simulink model "geometric_control_pertub"  (R2025b)
settings: Solver=ode45  StartTime=0.0  StopTime=t(end)  MaxStep=Ts  RelTol=1e-5
values from neighbouring files (symbols this model uses):
  A_tau = 0.002    [disturbances.m]    (also in scenarios_dist.m = K_dist * A_tau)
  A_wind = 0.1    [disturbances.m]    (also in scenarios_dist.m = K_dist * A_wind)
  Awind_0 = 0.5    [disturbances.m]    (also in scenarios_dist.m = K_dist * Awind_0)
  c_plant = 40/epsilon    (= 40)    [data.m]    (also in variation_params.m = scenarios(scen_idx, 2))
  Cd_eta = [0.08; 0.08; 0.05; 0.1; 0.1]    [disturbances.m]
  Cd_gamma = [0.01; 0.01; 0.01]    [disturbances.m]
  Cv_eta = [0.3; 0.3; 0.15; 0.4; 0.4]    [disturbances.m]
  Cv_gamma = [0.05; 0.05; 0.02]    [disturbances.m]
  dot_q_0 = -(dot_A_0 - (q_0' * dot_A_0) * q_0) / norm_A0    [trajectory_smooth.m]
  J = diag([Ixx, Iyy, Izz])    [data.m]
  k_plant = 1e5/epsilon^2    (= 100000)    [data.m]    (also in variation_params.m = scenarios(scen_idx, 1))
  kdq = 15    [control_params.m]
  kdw = 0.05    [disturbances.m]
  kO = 5    [control_params.m]
  kq = 50    [control_params.m]
  kr = 15    [control_params.m]
  kv = 15    [control_params.m]
  kx = 35    [control_params.m]
  L = 1    [data.m]
  l_0 = L + (m_L_plant * norm_A0) / (k_plant*m_sum_plant)    [trajectory_smooth.m]
  m_L = 0.5    [data.m]
  m_L_plant = m_L    (= 0.5)    [data.m]    (also in variation_params.m = scenarios(scen_idx, 3))
  m_q = 2    [data.m]
  Omega_0 = [0; 0; 0]    [trajectory_smooth.m]
  omega_0 = cross(q_0, dot_q_0)    [trajectory_smooth.m]
  omega_n_1 = 50    [control_params.m]
  omega_n_2 = 100    [control_params.m]
  omg_w = 0.8    [disturbances.m]
  q_0 = -A_0 / norm_A0    [trajectory_smooth.m]
  R_0 = [b1_0, b2_0, b3_0]    [trajectory_smooth.m]
  tau_phi_0 = 0.01    [disturbances.m]    (also in scenarios_dist.m = K_dist * tau_phi_0)
  tau_psi_0 = 0.005    [disturbances.m]    (also in scenarios_dist.m = K_dist * tau_psi_0)
  tau_theta_0 = 0.01    [disturbances.m]    (also in scenarios_dist.m = K_dist * tau_theta_0)
  vl_0 = dot_csi_d(:, 1)    [trajectory_smooth.m]
  xl_0 = csi_d(:, 1)    [trajectory_smooth.m]
  zeta_1 = 1    [control_params.m]
  zeta_2 = zeta_1    (= 1)    [control_params.m]
settings Model: Creator=emanu  LastModifiedBy=emanu

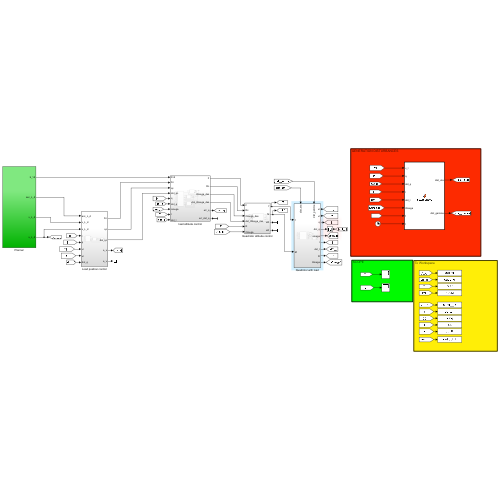
[thumbnail: Simulink's stored preview of the top-level diagram]
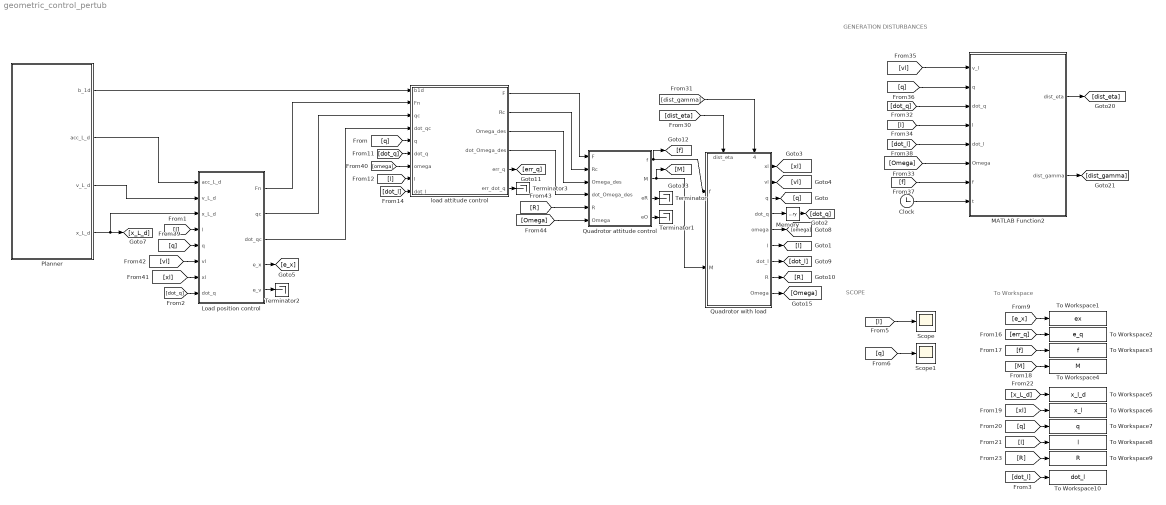
== system geometric_control_pertub ==
  note: GENERATION DISTURBANCES
  note: To Workspace
  note: SCOPE
  Clock : Clock
  Load position control : Subsystem
  MATLAB Function2 : MATLAB Function  TreatAsAtomicUnit=on
  Memory : Memory  InitialCondition=dot_q_0
  Planner : Subsystem
  Quadrotor attitude control : Subsystem
  Quadrotor with load : Subsystem
      settings: PortSchema="{\"entries\":[{\"content\":{\"sides\":[{\"content\":{\"connectorIds\":[\"In1\",\"In2\"]},\"type\":\"ConnectorPlacement.EquallySpacedRectSide\",\"uuid\":\"bde89180-b818-445b-bc24-a963d30a6ca2\"},{\"content\":{\"connectorIds\":[\"Out1\",\"Out2\",\"Out3\",\"Out4\",\"Out5\",\"Out6\",\"Out7\",\"Out8\",\"Out9\"],\"side\":\"RIGHT\"},\"type\":\"ConnectorPlacement.EquallySpacedRectSide\",\"uuid\":\"01dfe049-2eac-475a-b8e9-907eef5903e1\"},{\"content\":{\"connectorIds\":[\"In3\",\"In4\"],\"side\":\"TOP\"},\"type\":\"ConnectorPlacement.EquallySpacedRectSide\",\"uuid\":\"9cbb9b96-1170-48a0-bc43-4ca5d32b1acc\"}]},\"type\":\"ConnectorPlacement.EquallySpacedConnector\",\"uuid\":\"6cb2dbf7-60ad-42b8-8943-1cecbded3d22\"}],\"packageUris\":[\"http://schema.mathworks.com/mf0/Connector/R2020b\"],\"version\":\"1.0\"}"
  Scope : Scope
      settings: ActiveDisplayYMinimum=-1  ActiveDisplayYMaximum=1
  Scope1 : Scope
  Terminator{,1..3} (4 alike) : Terminator
  To Workspace1 : ToWorkspace  VariableName=ex  SaveFormat=Timeseries  SampleTime=-1
  To Workspace10 : ToWorkspace  VariableName=dot_l  SaveFormat=Timeseries  SampleTime=-1
  To Workspace2 : ToWorkspace  VariableName=e_q  SaveFormat=Timeseries  SampleTime=-1
  To Workspace3 : ToWorkspace  VariableName=f  SaveFormat=Timeseries  SampleTime=-1
  To Workspace4 : ToWorkspace  VariableName=M  SaveFormat=Timeseries  SampleTime=-1
  To Workspace5 : ToWorkspace  VariableName=x_l_d  SaveFormat=Timeseries  SampleTime=-1
  To Workspace6 : ToWorkspace  VariableName=x_l  SaveFormat=Timeseries  SampleTime=-1
  To Workspace7 : ToWorkspace  VariableName=q  SaveFormat=Timeseries  SampleTime=-1
  To Workspace8 : ToWorkspace  VariableName=l  SaveFormat=Timeseries  SampleTime=-1
  To Workspace9 : ToWorkspace  VariableName=R  SaveFormat=Timeseries  SampleTime=-1
  load attitude control : Subsystem
  wires:
  Quadrotor attitude control/1(f) -> [f], Quadrotor with load/1(f)
  Quadrotor attitude control/2(M) -> Quadrotor with load/2(M), [M]
  Quadrotor attitude control/3(eR) -> Terminator/1
  Quadrotor attitude control/4(eO) -> Terminator1/1
  load attitude control/1(F) -> Quadrotor attitude control/1(F)
  load attitude control/2(Rc) -> Quadrotor attitude control/2(Rc)
  load attitude control/3(Omega_des) -> Quadrotor attitude control/3(Omega_des)
  load attitude control/4(dot_Omega_des) -> Quadrotor attitude control/4(dot_Omega_des)
  Load position control/1(Fn) -> load attitude control/2(Fn)
  Load position control/2(qc) -> load attitude control/3(qc)
  Load position control/3(dot_qc) -> load attitude control/4(dot_qc)
  [l] -> Load position control/4(l)
  [dot_q] -> Load position control/8(dot_q)
  load attitude control/5(err_q) -> [err_q]
  load attitude control/6(err_dot_q) -> Terminator3/1
  Planner/1(b_1d) -> load attitude control/1(b1d)
  Planner/2(acc_L_d) -> Load position control/1(acc_L_d)
  Planner/3(v_L_d) -> Load position control/2(v_L_d)
  Planner/4(x_L_d) -> [x_L_d], Load position control/3(x_L_d)
  Quadrotor with load/6(l) -> [l]
  Quadrotor with load/5(omega) -> [omega]
  Quadrotor with load/3(q) -> [q]
  Quadrotor with load/1(xl) -> [xl]
  Quadrotor with load/2(vl) -> [vl]
  Load position control/4(e_x) -> [e_x]
  Load position control/5(e_v) -> Terminator2/1
  Memory/1 -> [dot_q]
  Quadrotor with load/4(dot_q) -> Memory/1
  [dot_q] -> load attitude control/6(dot_q)
  [l] -> load attitude control/8(l)
  Quadrotor with load/7(dot_l) -> [dot_l]
  [dot_l] -> load attitude control/9(dot_l)
  Quadrotor with load/8(R) -> [R]
  [e_x] -> To Workspace1/1
  [err_q] -> To Workspace2/1
  [f] -> To Workspace3/1
  [M] -> To Workspace4/1
  [x_L_d] -> To Workspace5/1
  [xl] -> To Workspace6/1
  [q] -> To Workspace7/1
  [l] -> To Workspace8/1
  [R] -> To Workspace9/1
  [l] -> Scope/1
  [q] -> Scope1/1
  Quadrotor with load/9(Omega) -> [Omega]
  MATLAB Function2/1(dist_eta) -> [dist_eta]
  MATLAB Function2/2(dist_gamma) -> [dist_gamma]
  [dist_eta] -> Quadrotor with load/3(dist_eta)
  [dist_gamma] -> Quadrotor with load/4(dist_gamma)
  [l] -> MATLAB Function2/4(l)
  [dot_q] -> MATLAB Function2/3(dot_q)
  [vl] -> MATLAB Function2/1(v_l)
  Clock/1 -> MATLAB Function2/8(t)
  [Omega] -> MATLAB Function2/6(Omega)
  [q] -> MATLAB Function2/2(q)
  [f] -> MATLAB Function2/7(f)
  [dot_l] -> MATLAB Function2/5(dot_l)
  [q] -> Load position control/5(q)
  [omega] -> load attitude control/7(omega)
  [xl] -> Load position control/7(xl)
  [vl] -> Load position control/6(vl)
  [R] -> Quadrotor attitude control/5(R)
  [Omega] -> Quadrotor attitude control/6(Omega)
  [q] -> load attitude control/5(q)
  [dot_l] -> To Workspace10/1

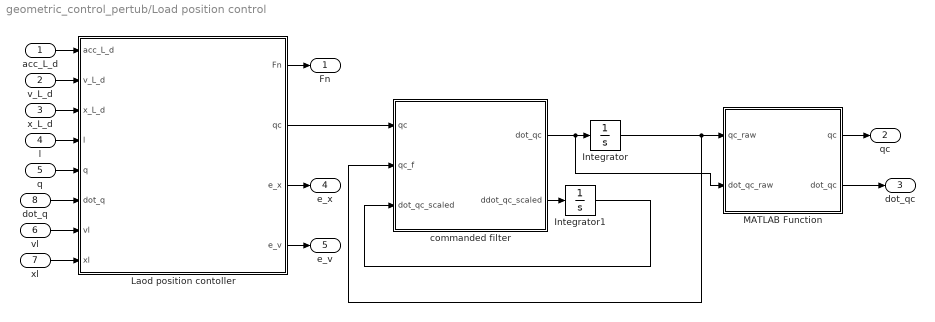
== system geometric_control_pertub/Load position control ==
  acc_L_d : Inport
  v_L_d : Inport  Port=2
  x_L_d : Inport  Port=3
  l : Inport  Port=4
  q : Inport  Port=5
  vl : Inport  Port=6
  xl : Inport  Port=7
  dot_q : Inport  Port=8
  Integrator : Integrator  InitialCondition=q_0
  Integrator1 : Integrator  InitialCondition=dot_q_0
  Laod position contoller : MATLAB Function  TreatAsAtomicUnit=on
  MATLAB Function : MATLAB Function  TreatAsAtomicUnit=on
  commanded filter : MATLAB Function  TreatAsAtomicUnit=on
  Fn : Outport
  qc : Outport  Port=2
  dot_qc : Outport  Port=3
  e_x : Outport  Port=4  VectorParamsAs1DForOutWhenUnconnected=off
  e_v : Outport  Port=5  VectorParamsAs1DForOutWhenUnconnected=off
  wires:
  acc_L_d/1 -> Laod position contoller/1(acc_L_d)
  v_L_d/1 -> Laod position contoller/2(v_L_d)
  x_L_d/1 -> Laod position contoller/3(x_L_d)
  l/1 -> Laod position contoller/4(l)
  q/1 -> Laod position contoller/5(q)
  vl/1 -> Laod position contoller/7(vl)
  xl/1 -> Laod position contoller/8(xl)
  Laod position contoller/1(Fn) -> Fn/1
  Laod position contoller/2(qc) -> commanded filter/1(qc)
  dot_q/1 -> Laod position contoller/6(dot_q)
  Laod position contoller/3(e_x) -> e_x/1
  Laod position contoller/4(e_v) -> e_v/1
  commanded filter/1(dot_qc) -> MATLAB Function/2(dot_qc_raw), Integrator/1
  Integrator/1 -> MATLAB Function/1(qc_raw), commanded filter/2(qc_f)
  commanded filter/2(ddot_qc_scaled) -> Integrator1/1
  Integrator1/1 -> commanded filter/3(dot_qc_scaled)
  MATLAB Function/1(qc) -> qc/1
  MATLAB Function/2(dot_qc) -> dot_qc/1

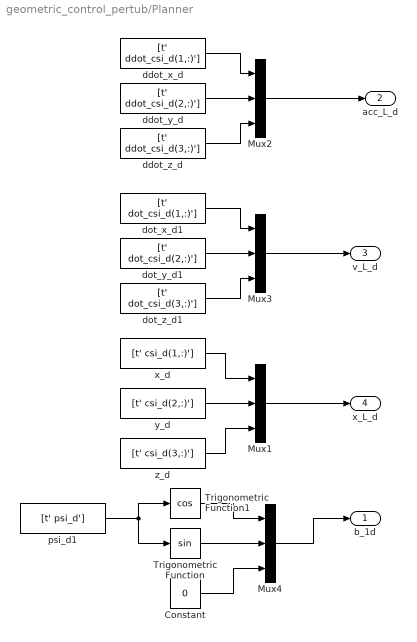
== system geometric_control_pertub/Planner ==
  Constant : Constant  Value=0
  Mux{1..4} (4 alike) : Mux  Inputs=3
  Trigonometric Function : Trigonometry
  Trigonometric Function1 : Trigonometry  Operator=cos
  ddot_x_d : FromWorkspace  VariableName=[t' ddot_csi_d(1,:)']  OutputAfterFinalValue=Holding final value
  ddot_y_d : FromWorkspace  VariableName=[t' ddot_csi_d(2,:)']  OutputAfterFinalValue=Holding final value
  ddot_z_d : FromWorkspace  VariableName=[t' ddot_csi_d(3,:)']  OutputAfterFinalValue=Holding final value
  dot_x_d1 : FromWorkspace  VariableName=[t' dot_csi_d(1,:)']  OutputAfterFinalValue=Holding final value
  dot_y_d1 : FromWorkspace  VariableName=[t' dot_csi_d(2,:)']  OutputAfterFinalValue=Holding final value
  dot_z_d1 : FromWorkspace  VariableName=[t' dot_csi_d(3,:)']  OutputAfterFinalValue=Holding final value
  psi_d1 : FromWorkspace  VariableName=[t' psi_d']  OutputAfterFinalValue=Holding final value
  x_d : FromWorkspace  VariableName=[t' csi_d(1,:)']  OutputAfterFinalValue=Holding final value
  y_d : FromWorkspace  VariableName=[t' csi_d(2,:)']  OutputAfterFinalValue=Holding final value
  z_d : FromWorkspace  VariableName=[t' csi_d(3,:)']  OutputAfterFinalValue=Holding final value
  b_1d : Outport
  acc_L_d : Outport  Port=2
  v_L_d : Outport  Port=3
  x_L_d : Outport  Port=4
  wires:
  y_d/1 -> Mux1/2
  z_d/1 -> Mux1/3
  x_d/1 -> Mux1/1
  ddot_y_d/1 -> Mux2/2
  ddot_z_d/1 -> Mux2/3
  ddot_x_d/1 -> Mux2/1
  Mux2/1 -> acc_L_d/1
  Mux1/1 -> x_L_d/1
  dot_y_d1/1 -> Mux3/2
  dot_z_d1/1 -> Mux3/3
  dot_x_d1/1 -> Mux3/1
  Mux3/1 -> v_L_d/1
  Mux4/1 -> b_1d/1
  Trigonometric Function/1 -> Mux4/2
  psi_d1/1 -> Trigonometric Function/1, Trigonometric Function1/1
  Trigonometric Function1/1 -> Mux4/1
  Constant/1 -> Mux4/3

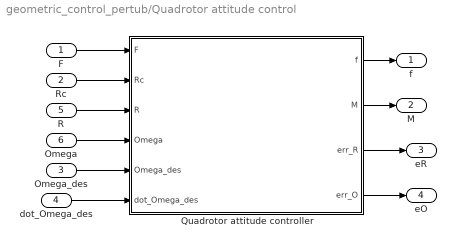
== system geometric_control_pertub/Quadrotor attitude control ==
  F : Inport
  Rc : Inport  Port=2
  Omega_des : Inport  Port=3
  dot_Omega_des : Inport  Port=4
  R : Inport  Port=5
  Omega : Inport  Port=6
  Quadrotor attitude controller : MATLAB Function  TreatAsAtomicUnit=on
  f : Outport
  M : Outport  Port=2
  eR : Outport  Port=3
  eO : Outport  Port=4
  wires:
  F/1 -> Quadrotor attitude controller/1(F)
  Quadrotor attitude controller/1(f) -> f/1
  Quadrotor attitude controller/2(M) -> M/1
  Quadrotor attitude controller/3(err_R) -> eR/1
  Quadrotor attitude controller/4(err_O) -> eO/1
  R/1 -> Quadrotor attitude controller/3(R)
  Omega/1 -> Quadrotor attitude controller/4(Omega)
  Omega_des/1 -> Quadrotor attitude controller/5(Omega_des)
  dot_Omega_des/1 -> Quadrotor attitude controller/6(dot_Omega_des)
  Rc/1 -> Quadrotor attitude controller/2(Rc)

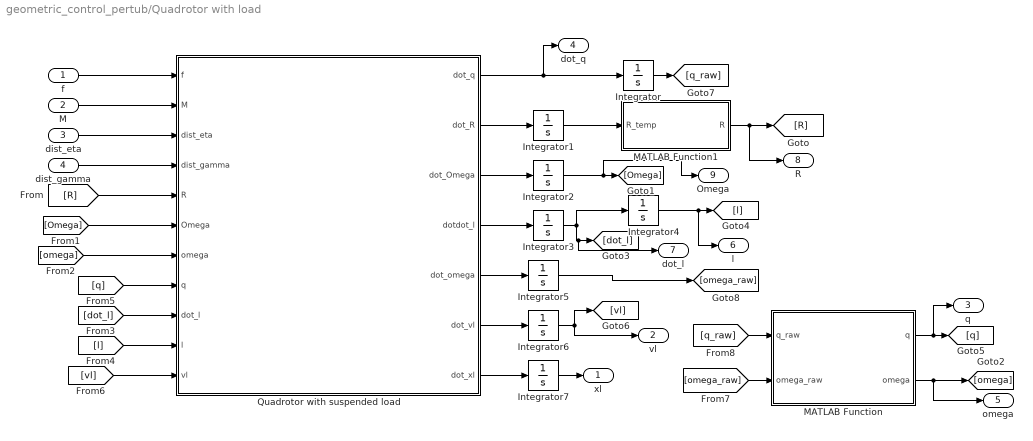
== system geometric_control_pertub/Quadrotor with load ==
  f : Inport
  M : Inport  Port=2
  dist_eta : Inport  Port=3
  dist_gamma : Inport  Port=4
  Integrator : Integrator  InitialCondition=q_0
  Integrator1 : Integrator  InitialCondition=R_0
  Integrator2 : Integrator  InitialCondition=Omega_0
  Integrator3 : Integrator
  Integrator4 : Integrator  InitialCondition=l_0
  Integrator5 : Integrator  InitialCondition=omega_0
  Integrator6 : Integrator  InitialCondition=vl_0
  Integrator7 : Integrator  InitialCondition=xl_0
  MATLAB Function : MATLAB Function  TreatAsAtomicUnit=on
  MATLAB Function1 : MATLAB Function  TreatAsAtomicUnit=on
  "Quadrotor with suspended load " : MATLAB Function  TreatAsAtomicUnit=on
  xl : Outport
  vl : Outport  Port=2
  q : Outport  Port=3
  dot_q : Outport  Port=4
  omega : Outport  Port=5
  l : Outport  Port=6
  dot_l : Outport  Port=7
  R : Outport  Port=8
  Omega : Outport  Port=9
  wires:
  f/1 -> "Quadrotor with suspended load "/1(f)
  M/1 -> "Quadrotor with suspended load "/2(M)
  "Quadrotor with suspended load "/1(dot_q) -> dot_q/1, Integrator/1
  "Quadrotor with suspended load "/2(dot_R) -> Integrator1/1
  Integrator1/1 -> MATLAB Function1/1(R_temp)
  MATLAB Function1/1(R) -> R/1, [R]
  [R] -> "Quadrotor with suspended load "/5(R)
  "Quadrotor with suspended load "/3(dot_Omega) -> Integrator2/1
  Integrator2/1 -> Omega/1, [Omega]
  [Omega] -> "Quadrotor with suspended load "/6(Omega)
  "Quadrotor with suspended load "/4(dotdot_l) -> Integrator3/1
  Integrator3/1 -> Integrator4/1, dot_l/1, [dot_l]
  "Quadrotor with suspended load "/5(dot_omega) -> Integrator5/1
  [omega] -> "Quadrotor with suspended load "/7(omega)
  [dot_l] -> "Quadrotor with suspended load "/9(dot_l)
  Integrator4/1 -> l/1, [l]
  [l] -> "Quadrotor with suspended load "/10(l)
  [q] -> "Quadrotor with suspended load "/8(q)
  "Quadrotor with suspended load "/6(dot_vl) -> Integrator6/1
  Integrator6/1 -> [vl], vl/1
  [vl] -> "Quadrotor with suspended load "/11(vl)
  "Quadrotor with suspended load "/7(dot_xl) -> Integrator7/1
  Integrator7/1 -> xl/1
  Integrator/1 -> [q_raw]
  Integrator5/1 -> [omega_raw]
  [omega_raw] -> MATLAB Function/2(omega_raw)
  [q_raw] -> MATLAB Function/1(q_raw)
  MATLAB Function/1(q) -> q/1, [q]
  MATLAB Function/2(omega) -> omega/1, [omega]
  dist_eta/1 -> "Quadrotor with suspended load "/3(dist_eta)
  dist_gamma/1 -> "Quadrotor with suspended load "/4(dist_gamma)

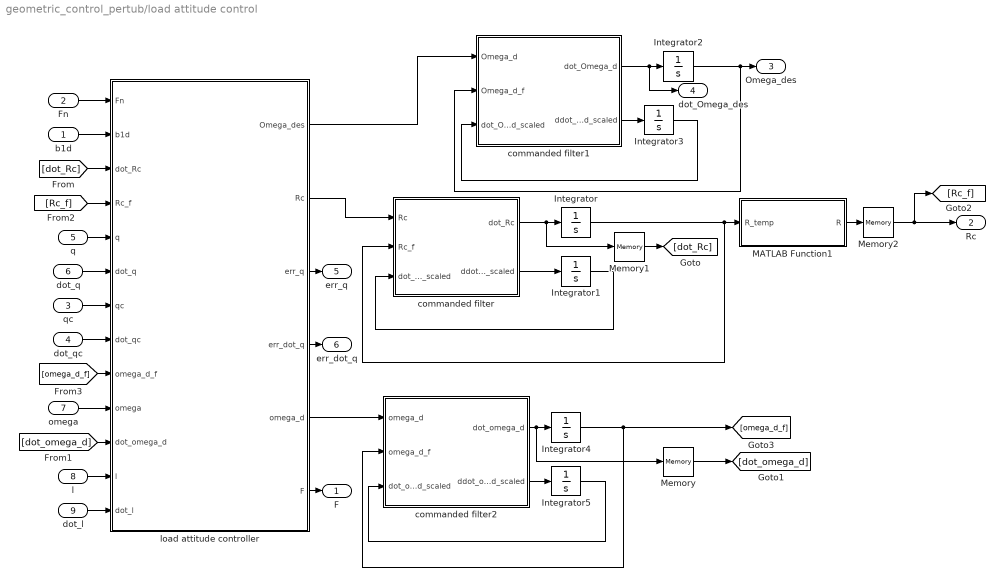
== system geometric_control_pertub/load attitude control ==
  b1d : Inport
  Fn : Inport  Port=2
  qc : Inport  Port=3
  dot_qc : Inport  Port=4
  q : Inport  Port=5
  dot_q : Inport  Port=6
  omega : Inport  Port=7
  l : Inport  Port=8
  dot_l : Inport  Port=9
  Integrator : Integrator  InitialCondition=R_0
  Integrator1 : Integrator  InitialCondition=zeros(3,3)
  Integrator2 : Integrator  InitialCondition=Omega_0
  Integrator3 : Integrator  InitialCondition=zeros(3,1)
  Integrator4 : Integrator  InitialCondition=omega_0
  Integrator5 : Integrator  InitialCondition=zeros(3,1)
  MATLAB Function1 : MATLAB Function  TreatAsAtomicUnit=on
  Memory : Memory  InitialCondition=zeros(3,1)
  Memory1 : Memory  InitialCondition=zeros(3,3)
  Memory2 : Memory  InitialCondition=R_0
  commanded filter : MATLAB Function  TreatAsAtomicUnit=on
  commanded filter1 : MATLAB Function  TreatAsAtomicUnit=on
  commanded filter2 : MATLAB Function  TreatAsAtomicUnit=on
  load attitude controller : MATLAB Function  TreatAsAtomicUnit=on
  F : Outport
  Rc : Outport  Port=2
  Omega_des : Outport  Port=3
  dot_Omega_des : Outport  Port=4
  err_q : Outport  Port=5  VectorParamsAs1DForOutWhenUnconnected=off
  err_dot_q : Outport  Port=6
  wires:
  load attitude controller/2(Rc) -> commanded filter/1(Rc)
  [dot_Rc] -> load attitude controller/3(dot_Rc)
  Integrator5/1 -> commanded filter2/3(dot_omega_d_scaled)
  [dot_omega_d] -> load attitude controller/11(dot_omega_d)
  qc/1 -> load attitude controller/7(qc)
  dot_qc/1 -> load attitude controller/8(dot_qc)
  q/1 -> load attitude controller/5(q)
  dot_q/1 -> load attitude controller/6(dot_q)
  omega/1 -> load attitude controller/10(omega)
  l/1 -> load attitude controller/12(l)
  dot_l/1 -> load attitude controller/13(dot_l)
  load attitude controller/6(F) -> F/1
  b1d/1 -> load attitude controller/2(b1d)
  Fn/1 -> load attitude controller/1(Fn)
  load attitude controller/3(err_q) -> err_q/1
  load attitude controller/4(err_dot_q) -> err_dot_q/1
  commanded filter/1(dot_Rc) -> Memory1/1, Integrator/1
  Integrator1/1 -> commanded filter/3(dot_Rc_scaled)
  Integrator/1 -> commanded filter/2(Rc_f), MATLAB Function1/1(R_temp)
  commanded filter/2(ddot_Rc_scaled) -> Integrator1/1
  commanded filter2/2(ddot_omega_d_scaled) -> Integrator5/1
  commanded filter2/1(dot_omega_d) -> Memory/1, Integrator4/1
  load attitude controller/5(omega_d) -> commanded filter2/1(omega_d)
  commanded filter1/1(dot_Omega_d) -> dot_Omega_des/1, Integrator2/1
  commanded filter1/2(ddot_Omega_d_scaled) -> Integrator3/1
  Integrator2/1 -> Omega_des/1, commanded filter1/2(Omega_d_f)
  Integrator3/1 -> commanded filter1/3(dot_Omega_d_scaled)
  load attitude controller/1(Omega_des) -> commanded filter1/1(Omega_d)
  [Rc_f] -> load attitude controller/4(Rc_f)
  Integrator4/1 -> [omega_d_f], commanded filter2/2(omega_d_f)
  [omega_d_f] -> load attitude controller/9(omega_d_f)
  MATLAB Function1/1(R) -> Memory2/1
  Memory2/1 -> Rc/1, [Rc_f]
  Memory1/1 -> [dot_Rc]
  Memory/1 -> [dot_omega_d]

== matlab function geometric_control_pertub/Load position control/Laod position contoller ==
  data: acc_L_d input size=3; Fn output size=3; v_L_d input size=3; x_L_d input size=3; l input size=1; q input size=3; dot_q input size=3; vl input size=3; xl input size=3; qc output size=3; m_q parameter; m_L parameter; e_x output size=3; e_v output size=3; kx parameter; kv parameter
function [Fn,qc,e_x,e_v] = fcn(acc_L_d,v_L_d,x_L_d,l,q,dot_q,vl,xl,m_q, m_L,kx, kv)

g=9.81;
m_sum=m_q+m_L;
e_x=xl-x_L_d;
e_v=vl-v_L_d;

k_x =kx;
k_v = kv;

A=-k_x*e_x-k_v*e_v+m_sum*(acc_L_d+g*[0;0;1])+m_q*l*(dot_q'*dot_q)*q;
if norm(A)>1e-6
     qc=-A/norm(A);
else
    qc = [0; 0; -1];
end
Fn = (A' * q) * q;
end

== matlab function geometric_control_pertub/Quadrotor with load/MATLAB Function1 ==
  data: R_temp input; R output
function R = fcn(R_temp)
    [U,S,V] = svd(R_temp);
    sigma = det(U*V');
    S_ = diag([1 1 sigma]);

    R = U*S_*V';
end

== matlab function geometric_control_pertub/Quadrotor with load/MATLAB Function ==
  data: q_raw input; q output; omega_raw input; omega output
function [q, omega] = fcn(q_raw, omega_raw)
   
    q_raw = q_raw(:);
    omega_raw = omega_raw(:);

    
    q = q_raw / norm(q_raw);

  
    omega = omega_raw - (q' * omega_raw) * q;
end

== matlab function geometric_control_pertub/Load position control/commanded filter ==
  data: qc input; dot_qc output; qc_f input; dot_qc_scaled input; ddot_qc_scaled output; zeta_1 parameter; omega_n_1 parameter
function [dot_qc, ddot_qc_scaled] = fcn(qc, qc_f, dot_qc_scaled, zeta_1, omega_n_1)
    dot_qc = omega_n_1 * dot_qc_scaled;
    ddot_qc_scaled = -2 * zeta_1 * omega_n_1 * dot_qc_scaled - omega_n_1 * (qc_f - qc);
end

== matlab function geometric_control_pertub/load attitude control/commanded filter ==
  data: Rc input; dot_Rc output; Rc_f input; dot_Rc_scaled input; zeta_2 parameter; ddot_Rc_scaled output; omega_n_2 parameter
function [dot_Rc, ddot_Rc_scaled] = fcn(Rc, Rc_f, dot_Rc_scaled, zeta_2, omega_n_2)
    dot_Rc = omega_n_2 * dot_Rc_scaled;
    ddot_Rc_scaled = -2 * zeta_2 * omega_n_2 * dot_Rc_scaled - omega_n_2 * (Rc_f - Rc);
end

== matlab function geometric_control_pertub/load attitude control/commanded filter1 ==
  data: Omega_d input; dot_Omega_d output; Omega_d_f input; dot_Omega_d_scaled input; zeta_2 parameter; ddot_Omega_d_scaled output; omega_n_2 parameter
function [dot_Omega_d, ddot_Omega_d_scaled] = fcn(Omega_d, Omega_d_f, dot_Omega_d_scaled, zeta_2, omega_n_2)
    dot_Omega_d = omega_n_2 * dot_Omega_d_scaled;
    ddot_Omega_d_scaled = -2 * zeta_2 * omega_n_2 * dot_Omega_d_scaled - omega_n_2 * (Omega_d_f - Omega_d);
end

== matlab function geometric_control_pertub/load attitude control/commanded filter2 ==
  data: omega_d input; dot_omega_d output; omega_d_f input; dot_omega_d_scaled input; zeta_2 parameter; ddot_omega_d_scaled output; omega_n_2 parameter
function [dot_omega_d, ddot_omega_d_scaled] = fcn(omega_d, omega_d_f, dot_omega_d_scaled, zeta_2, omega_n_2)
    dot_omega_d = omega_n_2 * dot_omega_d_scaled;
    ddot_omega_d_scaled = -2 * zeta_2 * omega_n_2 * dot_omega_d_scaled - omega_n_2 * (omega_d_f - omega_d);
end

== matlab function geometric_control_pertub/load attitude control/MATLAB Function1 ==
  data: R_temp input; R output
function R = fcn(R_temp)
    [U,S,V] = svd(R_temp);
    sigma = det(U*V');
    S_ = diag([1 1 sigma]);

    R = U*S_*V';
end

== matlab function geometric_control_pertub/Load position control/MATLAB Function ==
  data: qc_raw input; qc output; dot_qc_raw input; dot_qc output
function [qc, dot_qc] = S2_projection(qc_raw, dot_qc_raw)
   
    norm_qc = norm(qc_raw);
    if norm_qc > 1e-6
        qc = qc_raw / norm_qc;
    else
        qc = [0; 0; -1]; 
    end
    dot_qc = dot_qc_raw - (qc' * dot_qc_raw) * qc;
end

== matlab function geometric_control_pertub/MATLAB Function2 ==
  data: v_l input size=3; q input size=3; dist_eta output size=5; dist_gamma output size=3; dot_q input size=3; l input size=1; dot_l input size=1; Omega input size=3; f input; t input; omg_w parameter size=1; A_wind parameter size=1; Awind_0 parameter size=1; kdw parameter size=1; Cv_eta parameter size=5; Cv_gamma parameter size=3; Cd_eta parameter size=5; Cd_gamma parameter size=3; tau_phi_0 parameter size=1; tau_psi_0 parameter size=1; A_tau parameter size=1; tau_theta_0 parameter
function [dist_eta, dist_gamma] = disturbances(...
    v_l, q, dot_q, l, dot_l, Omega, f, t, omg_w, A_wind, Awind_0, kdw, ...
    Cv_eta, Cv_gamma, Cd_eta, Cd_gamma, tau_phi_0, tau_psi_0, A_tau, tau_theta_0)

v_q = v_l - dot_l * q - l * dot_q;
cos_beta = max(sqrt(q(1)^2 + q(3)^2), 0.01); 
d_beta  = dot_q(2) / cos_beta;
d_alpha = (q(3)*dot_q(1) - q(1)*dot_q(3)) / (q(1)^2 + q(3)^2);


eta_dot   = [v_q; d_alpha; d_beta];
gamma_dot = Omega;
Fwind_x = Awind_0 + A_wind * sin(omg_w * t);
Fwind_y = 0.5 * Awind_0 + A_wind * cos(0.7 * omg_w * t);
F_downwash_z = kdw * f;


dist_eta_0 = [Fwind_x; Fwind_y; F_downwash_z; 0; 0];
dist_gamma_0 = [
    tau_phi_0   + A_tau * sin(0.6 * t);
    tau_theta_0 + A_tau * cos(0.4 * t);
    tau_psi_0
];

dist_eta_1   = Cv_eta .* eta_dot;
dist_gamma_1 = Cv_gamma .* gamma_dot;

dist_eta_2   = Cd_eta .* (eta_dot .* abs(eta_dot));
dist_gamma_2 = Cd_gamma .* (gamma_dot .* abs(gamma_dot));

dist_eta   = dist_eta_0 + dist_eta_1 + dist_eta_2;
dist_gamma = dist_gamma_0 + dist_gamma_1 + dist_gamma_2;

end

== matlab function geometric_control_pertub/Quadrotor attitude control/Quadrotor attitude controller ==
  data: F input size=3; f output; M output size=3; Rc input size=[3,3]; R input size=[3,3]; Omega input size=3; Omega_des input size=3; err_R output size=3; err_O output size=3; dot_Omega_des input size=3; J parameter; kr parameter; kO parameter
function [f,M,err_R,err_O] = Quad_Att_controller(F,Rc,R,Omega,Omega_des, dot_Omega_des,J,kr, kO)

k_R =kr; %4.1;
k_O =kO; %0.47;
epn = 0.7;

%compute error 
err_R = wedge((Rc'*R-R'*Rc))/2;

err_O=Omega-R'*Rc*Omega_des;

%Compute M and f
M=-(1/epn^2)*k_R*err_R-(1/epn)*k_O*err_O+skew(Omega)*J*Omega-J*(skew(Omega)*R'*Rc*Omega_des-R'*Rc*dot_Omega_des);


f=F'*(R*[0;0;1]);

end

function S = skew(v)
if(numel(v)~= 1)
S= [0 -v(3) v(2); 
    v(3) 0 -v(1);
    -v(2) v(1) 0];
else
S= zeros(3);
end
end

function v = wedge(S)
v1 = S(3,2);
v2 = S(1,3);
v3 = S(2,1);
v = [v1 v2 v3]';
end

== matlab function geometric_control_pertub/Quadrotor with load/Quadrotor with suspended load  ==
  data: dot_q output size=3; dot_R output size=[3,3]; f input size=1; M input size=3; dist_eta input; dist_gamma input; R input size=[3,3]; dot_Omega output size=3; Omega input size=3; omega input size=3; q input size=3; dot_l input size=1; l input size=1; vl input size=3; J parameter; m_q parameter; m_L_plant parameter; k_plant parameter; c_plant parameter; dotdot_l output size=1; dot_omega output size=3; dot_vl output size=3; dot_xl output size=3; L parameter
function [dot_q, dot_R, dot_Omega, dotdot_l, dot_omega, dot_vl, dot_xl] = dynamics(...
    f, M, dist_eta, dist_gamma, R, Omega, omega, q, dot_l, l, vl, J, m_q, m_L_plant, k_plant, c_plant, L)

m_sum = m_q + m_L_plant;
m_t   = m_sum / (m_q * m_L_plant);
g     = 9.81;

F_thrust = f * R * [0; 0; 1];

F_total  = F_thrust - dist_eta(1:3);

M_total   = M - dist_gamma;
dot_Omega = J \ (M_total - skew(Omega) * J * Omega);
dot_R     = R * skew(Omega);

dist_alpha = dist_eta(4);
dist_beta  = dist_eta(5);

den2 = q(1)^2 + q(3)^2;
den  = max(sqrt(den2), 0.01); 
den2 = max(den2, 0.0001);     

dist_omega_x = -dist_alpha * (q(1)*q(2)/den2) - dist_beta * (q(3)/den);
dist_omega_y =  dist_alpha;
dist_omega_z = -dist_alpha * (q(2)*q(3)/den2) + dist_beta * (q(1)/den);

dist_omega = [dist_omega_x; dist_omega_y; dist_omega_z];

dot_q = skew(omega) * q;
dotdot_l = l * (dot_q' * dot_q) + m_t * k_plant * (L - l) - m_t * c_plant * dot_l - (1 / m_q) * (q' * F_total);
dot_omega = -1 / (m_q * l) * skew(q) * F_total - (2 / l) * dot_l * omega - dist_omega;

H = (m_q * dotdot_l + q' * F_total - m_q * l * (dot_q' * dot_q)) * q;
dot_vl = (H / m_sum) - g * [0; 0; 1];
dot_xl = vl;

end

function S = skew(v)
if numel(v) ~= 1
    S = [ 0     -v(3)   v(2); 
         v(3)    0     -v(1);
        -v(2)   v(1)    0   ];
else
    S = zeros(3);
end
end

== matlab function geometric_control_pertub/load attitude control/load attitude controller ==
  data: Fn input size=3; b1d input size=3; Omega_des output size=3; Rc output size=[3,3]; dot_Rc input size=[3,3]; Rc_f input; q input size=3; dot_q input size=3; qc input size=3; dot_qc input size=3; omega_d_f input; omega input size=3; err_q output size=3; err_dot_q output size=3; omega_d output size=3; F output size=3; dot_omega_d input size=3; l input size=1; dot_l input size=1; m_q parameter; kq parameter; kdq parameter
function [Omega_des,Rc,err_q,err_dot_q,omega_d,F] = fcn(Fn,b1d,dot_Rc,Rc_f,q,dot_q,qc,dot_qc,omega_d_f,omega,dot_omega_d,l,dot_l,m_q,kq, kdq)

q_hat = skew(q);
err_q= (q_hat * q_hat) * qc;

err_dot_q=dot_q-skew(omega_d_f)*q;

k_q = kq;
k_q_dot = kdq;
F_pd= -k_q*err_q-k_q_dot*err_dot_q;

omega_d=skew(qc)*dot_qc;
dot_omega_d_ = dot_omega_d - (qc' * dot_omega_d) * qc;
F_ff=m_q*l*(q'*omega_d)*omega+m_q*l*skew(dot_omega_d_)*q+2*m_q*dot_l*skew(omega)*q;
F=Fn-F_pd-F_ff;
norm_F = norm(F);

if norm_F > 1e-6 
    b3c = F / norm_F;
else
    b3c = [0; 0; 1]; 
end
S_b3c = skew(b3c);
const=1e-6;
b1c = - (S_b3c * S_b3c * b1d) / (norm(S_b3c * b1d) + const);

r2=skew(b3c)*b1c;
Rc=[b1c r2 b3c];

M = Rc_f' * dot_Rc;
M_skew = 0.5 * (M - M');
Omega_des = wedge(M_skew);

end


function S = skew(v)

S = [  0,   -v(3),  v(2); 
     v(3),     0,  -v(1);
    -v(2),   v(1),    0];
end

function v = wedge(S)

v = [S(3,2); S(1,3); S(2,1)];
end
